simulink model "MotorModeloFFB"  (R2021a)
settings: Solver=VariableStepAuto  StartTime=0.0  StopTime=t_fin  MaxStep=1e-5  RelTol=1e-3
InitFcn:
  | Cargar_Ensayo3
values from neighbouring files (symbols this model uses):
  B = p0(2)    [DC_Motor.m]    (also in Parametros_Motor_FFB.m = pm_.B)
  J = p0(1)    [DC_Motor.m]    (also in Parametros_Motor_FFB.m = pm_.J)
  Ka = p0(3)    [DC_Motor.m]    (also in Parametros_Motor_FFB.m = pm_.Ka)
  Km = p0(4)    [DC_Motor.m]    (also in Parametros_Motor_FFB.m = 0.0225)
  L = p0(6)    [DC_Motor.m]    (also in Parametros_Motor_FFB.m = pm_.L)
  R = R_motor    [Ajuste_Modelo_Captura.m]    (also in Capturar_Escalon.m; Cargar_Ensayo3.m; DC_Motor.m = p0(5); Parametros_Motor_FFB.m = pm_.R)
  Tc = pm_.Tc    [Parametros_Motor_FFB.m]
  Ts_data = 1e-5    (= 1e-05)    [Cargar_Ensayo3.m]
  Vm = 9    [Parametros_Motor_FFB.m]    (also in Regresion_Modelo.m = 3.57)
  w_tc = 1    [Parametros_Motor_FFB.m]
libraries: cstblocks x2
settings Model: Creator=Sergio  LastModifiedBy=norie
settings SolverCC: AlgebraicLoopSolver=TrustRegion
settings DataIOCC: ReturnWorkspaceOutputs=off
settings DebuggingCC: SFMachineParentedDataDiag=warning  ArithmeticOperatorsInVariantConditions=warning
settings SFSimCC: SimUseLocalCustomCode=off  CustomCodeUndefinedFunction=UseInterfaceOnly
settings RTWCC: RTWUseLocalCustomCode=off

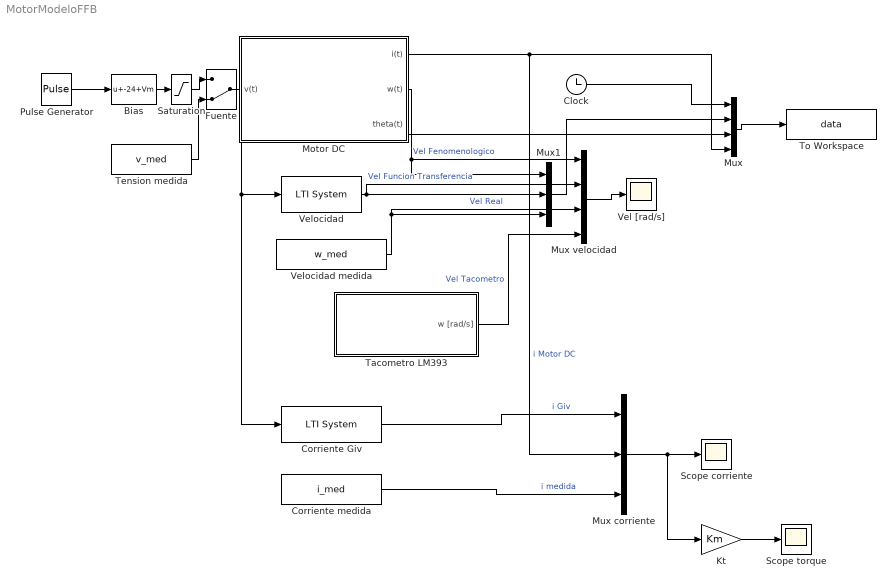
== system MotorModeloFFB ==
  Bias : Bias  Bias=-24+Vm
  Clock : Clock
  Corriente Giv : cstblocks/LTI System  sys=Giv  IC=[]
  Corriente medida : FromWorkspace  VariableName=i_med  OutputAfterFinalValue=Holding final value
  Fuente : ManualSwitch  CurrentSetting=0
  Kt : Gain  Gain=Km
  Motor DC : Subsystem
  Mux : Mux
  Mux corriente : Mux  Inputs=3
  Mux velocidad : Mux
  Mux1 : Mux  Inputs=3
  Pulse Generator : DiscretePulseGenerator  PulseType=Time based  Amplitude=24  Period=4  PulseWidth=50  PhaseDelay=2
  Saturation : Saturate  UpperLimit=24  LowerLimit=0
  Scope corriente : Scope
  Scope torque : Scope
  Tacometro LM393 : Subsystem
  Tension medida : FromWorkspace  VariableName=v_med  Interpolate=off  OutputAfterFinalValue=Holding final value
  To Workspace : ToWorkspace  VariableName=data  SampleTime=Ts_data
  Vel [rad/s] : Scope
  Velocidad : cstblocks/LTI System  sys=Gwv  IC=[]
  Velocidad medida : FromWorkspace  VariableName=w_med  OutputAfterFinalValue=Holding final value
  wires:
  Motor DC/2(w(t)) -> Mux1/1, Mux velocidad/1  "Vel Fenomenologico"
  Velocidad/1 -> Mux1/2, Mux velocidad/2  "Vel Funcion Transferencia"
  Bias/1 -> Saturation/1
  Mux/1 -> To Workspace/1
  Clock/1 -> Mux/1
  Mux1/1 -> Mux/2
  Pulse Generator/1 -> Bias/1
  Motor DC/1(i(t)) -> Mux/4, Mux corriente/2  "i Motor DC"
  Corriente Giv/1 -> Mux corriente/1  "i Giv"
  Corriente medida/1 -> Mux corriente/3  "i medida"
  Mux corriente/1 -> Scope corriente/1, Kt/1
  Kt/1 -> Scope torque/1
  Saturation/1 -> Fuente/1
  Tension medida/1 -> Fuente/2
  Fuente/1 -> Velocidad/1, Corriente Giv/1, Mux/3, Motor DC/1(v(t))
  Tacometro LM393/1(w [rad/s]) -> Mux velocidad/4  "Vel Tacometro"
  Mux velocidad/1 -> Vel [rad/s]/1
  Velocidad medida/1 -> Mux1/3, Mux velocidad/3  "Vel Real"

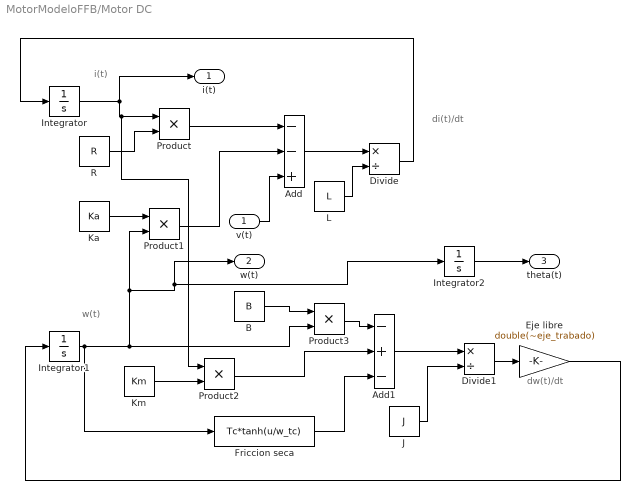
== system MotorModeloFFB/Motor DC ==
  note: i(t)
  note: w(t)
  note: di(t)/dt
  note: dw(t)/dt
  v(t) : Inport
  Add : Sum  Inputs=--+
  Add1 : Sum  Inputs=-+-
  B : Constant  Value=B
  Divide : Product  Inputs=*/
  Divide1 : Product  Inputs=*/
  Eje libre : Gain  Gain=double(~eje_trabado)
  Friccion seca : Fcn  Expr=Tc*tanh(u/w_tc)
  Integrator : Integrator
  Integrator1 : Integrator
  Integrator2 : Integrator
  J : Constant  Value=J
  Ka : Constant  Value=Ka
  Km : Constant  Value=Km
  L : Constant  Value=L
  Product{,1..3} (4 alike) : Product
  R : Constant  Value=R
  i(t) : Outport  VectorParamsAs1DForOutWhenUnconnected=off
  w(t) : Outport  Port=2  VectorParamsAs1DForOutWhenUnconnected=off
  theta(t) : Outport  Port=3  VectorParamsAs1DForOutWhenUnconnected=off
  wires:
  Divide/1 -> Integrator/1
  Integrator/1 -> i(t)/1, Product2/1, Product/1
  Integrator1/1 -> Product3/2, w(t)/1, Integrator2/1, Product1/2, Friccion seca/1
  R/1 -> Product/2
  Add1/1 -> Divide1/1
  v(t)/1 -> Add/3
  Ka/1 -> Product1/1
  J/1 -> Divide1/2
  Product3/1 -> Add1/1
  Product1/1 -> Add/2
  Add/1 -> Divide/1
  Product/1 -> Add/1
  L/1 -> Divide/2
  Integrator2/1 -> theta(t)/1
  B/1 -> Product3/1
  Km/1 -> Product2/2
  Product2/1 -> Add1/2
  Friccion seca/1 -> Add1/3
  Divide1/1 -> Eje libre/1
  Eje libre/1 -> Integrator1/1

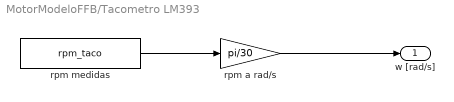
== system MotorModeloFFB/Tacometro LM393 ==
  rpm a rad/s : Gain  Gain=pi/30
  rpm medidas : FromWorkspace  VariableName=rpm_taco  OutputAfterFinalValue=Holding final value
  w [rad/s] : Outport
  wires:
  rpm medidas/1 -> rpm a rad/s/1
  rpm a rad/s/1 -> w [rad/s]/1
